simulink model "state_estimation"  (R2024b)
settings: Solver=VariableStepAuto  StartTime=0.0  StopTime=10.0  RelTol=1e-3
values from neighbouring files (symbols this model uses):
  A = [0 1;-1/T^2 -2*c/T]    [steady_state_model.m]
  A_plant = [0 1;-1/T_plant^2 -2*c_plant/T_plant]    [steady_state_model.m]
  B = [0;K/T^2]    [steady_state_model.m]
  B_plant = [0;K_plant/T_plant^2]    [steady_state_model.m]
  C = [1 0]    [steady_state_model.m]
  C_plant = [1 0]    [steady_state_model.m]
  D = 0    [steady_state_model.m]
  D_plant = 0    [steady_state_model.m]
  Lobs = place(Ap',Cp',obsPoles)'    [steady_state_model.m]
settings Model: Creator=zhangyutong  LastModifiedBy=zhangyutong

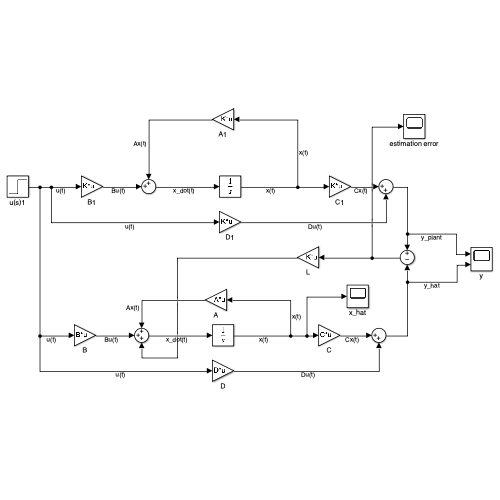
[thumbnail: Simulink's stored preview of the top-level diagram]
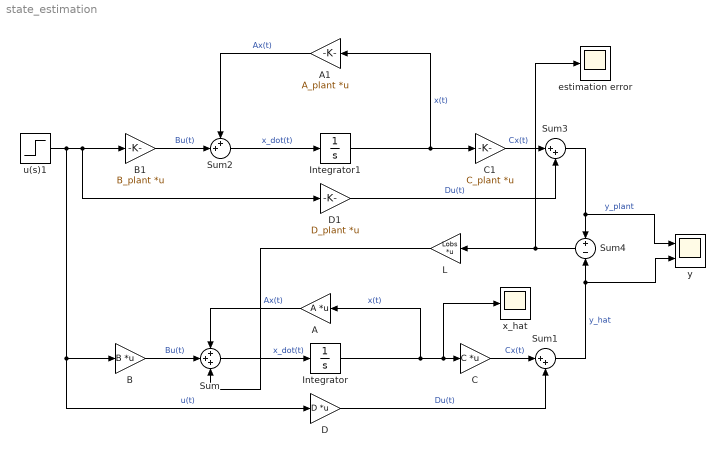
== system state_estimation ==
  A : Gain  Gain=A  Multiplication=Matrix(K*u)
  A1 : Gain  Gain=A_plant  Multiplication=Matrix(K*u)
  B : Gain  Gain=B  Multiplication=Matrix(K*u)
  B1 : Gain  Gain=B_plant  Multiplication=Matrix(K*u)
  C : Gain  Gain=C  Multiplication=Matrix(K*u)
  C1 : Gain  Gain=C_plant  Multiplication=Matrix(K*u)
  D : Gain  Gain=D  Multiplication=Matrix(K*u)
  D1 : Gain  Gain=D_plant  Multiplication=Matrix(K*u)
  Integrator : Integrator  InitialCondition=[0;0]
  Integrator1 : Integrator  InitialCondition=[0;0]
  L : Gain  Gain=Lobs  Multiplication=Matrix(K*u)
  Sum : Sum  Inputs=+++
  Sum1 : Sum  Inputs=|++
  Sum2 : Sum  Inputs=++|
  Sum3 : Sum  Inputs=|++
  Sum4 : Sum  Inputs=+|-
  estimation error : Scope
  u(s)1 : Step  Time=0  SampleTime=0
  x_hat : Scope
  y : Scope  NumInputPorts=2
  wires:
  B/1 -> Sum/2  "Bu(t)"
  Sum/1 -> Integrator/1  "x_dot(t)"
  Integrator/1 -> A/1, x_hat/1, C/1  "x(t)"
  A/1 -> Sum/1  "Ax(t)"
  Sum1/1 -> y/2, Sum4/2  "y_hat"
  C/1 -> Sum1/1  "Cx(t)"
  D/1 -> Sum1/2  "Du(t)"
  Sum2/1 -> Integrator1/1  "x_dot(t)"
  Integrator1/1 -> A1/1, C1/1  "x(t)"
  u(s)1/1 -> D/1, B/1, D1/1, B1/1  "u(t)"
  A1/1 -> Sum2/1  "Ax(t)"
  Sum3/1 -> Sum4/1, y/1  "y_plant"
  B1/1 -> Sum2/2  "Bu(t)"
  C1/1 -> Sum3/1  "Cx(t)"
  D1/1 -> Sum3/2  "Du(t)"
  Sum4/1 -> estimation error/1, L/1
  L/1 -> Sum/3
